simulink library "filters_lib"  (R2018b)
settings: Solver=VariableStepAuto  StartTime=0.0  StopTime=10.0  RelTol=1e-3
undefined symbols (not defined in the file or in its folder): DiscIntNeverNeededParam, u_Trim
libraries: quatAttitudeController_lib x1
settings Model: Creator=Ybeyer  LastModifiedBy=yannic
settings DebuggingCC: LibraryContextMissingDiagnostic=none
settings SFSimCC: SimUseLocalCustomCode=off
settings RTWCC: RTWUseLocalCustomCode=off
settings CodeAppCC: StateflowObjectComments=on

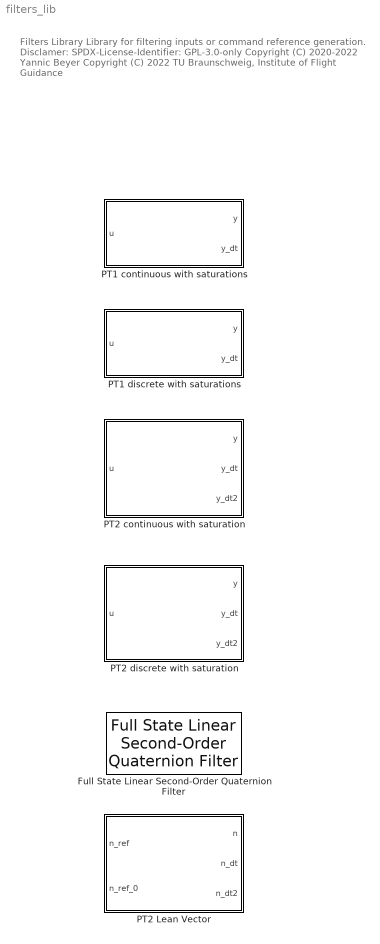
== system filters_lib ==
  note: Filters Library
      |
      | Library for filtering inputs or command reference generation.
      |
      | Disclamer:
      | SPDX-License-Identifier: GPL-3.0-only
      |
      | Copyright (C) 2020-2022 Yannic Beyer
      | Copyright (C) 2022 TU Braunschweig, Institute of Flight Guidance
  Full State Linear Second-Order Quaternion Filter : quatAttitudeController_lib/Full State Linear Second-Order Quaternion Filter  omega_0=15  D=1  q_0=[1; 0; 0; 0]  omega_Kb_0=[0; 0; 0]
      settings: SourceProductName=LADAC
  PT1 continuous with saturations : Subsystem  mask{T=1, x_max=inf, x_min=-inf, x_dt_max=inf, x_dt_min=-inf, x_init=0}
      mask prompts: T "Time constant"; x_max "Maximum output"; x_min "Minimum output"; x_dt_max "Maximum output_rate"; x_dt_min "Minimum output rate"; x_init "Initial output"
  PT1 discrete with saturations : Subsystem  mask{T=1, x_max=inf, x_min=-inf, x_dt_max=inf, x_dt_min=-inf, x_init=u_Trim}
      mask prompts: T "Time constant"; x_max "Maximum output"; x_min "Minimum output"; x_dt_max "Maximum output rate"; x_dt_min "Minimum output rate"; x_init "Initial output"
  PT2 Lean Vector : Subsystem  mask{omega=1, d=1, x_dt2_max=inf, x_dt2_min=-inf, x_dt_max=inf, x_dt_min=-inf, x_max=inf, x_min=-inf, x_init=0, x_dt_init=0}
      mask prompts: omega "Natural frequency"; d "Damping ratio"; x_dt2_max "Maximum acceleration"; x_dt2_min "Minimum acceleration"; x_dt_max "Maximum rate"; x_dt_min "Minimum rate"; x_max "Maximum position"; x_min "Minimum position"; x_init "Initial position"; x_dt_init "Initial rate"
      mask DialogControl DescGroupVar Prompt: 2nd Order Reduced Attitude Reference Model
      mask DialogControl DescTextVar Prompt: The lean vector is filtered by a second order low-pass filter. A unit vector output is assured. Moreover, the derivatives are also adjusted to match with the output unit vector.
  PT2 continuous with saturation : Subsystem  mask{omega=0.7, d=1, x_dt2_max=inf, x_dt2_min=-inf, x_dt_max=inf, x_dt_min=-inf, x_max=inf, x_min=-inf, x_init=0, x_dt_init=0}
      mask prompts: omega "Natural frequency"; d "Damping ratio"; x_dt2_max "Maximum acceleration"; x_dt2_min "Minimum acceleration"; x_dt_max "Maximum rate"; x_dt_min "Minimum rate"; x_max "Maximum position"; x_min "Minimum position"; x_init "Initial position"; x_dt_init "Initial rate"
  PT2 discrete with saturation : Subsystem  mask{param_src=internal, omega=1, d=0.7, x_dt2_max=inf, x_dt2_min=-inf, x_dt_max=inf, x_dt_min=-inf, x_max=inf, x_min=-inf, y_0_src=internal, x_init=0, y_dt_0_src=internal, x_dt_init=0, is_y_dt_checked=on, is_y_dt2_checked=on}
      mask prompts: param_src "Parameter source"; omega "Natural frequency"; d "Damping ratio"; x_dt2_max "Maximum acceleration"; x_dt2_min "Minimum acceleration"; x_dt_max "Maximum rate"; x_dt_min "Minimum rate"; x_max "Maximum position"; x_min "Minimum position"; y_0_src "Initial position source:"; x_init "Initial position"; y_dt_0_src "Initial velocity source:"; x_dt_init "Initial rate"; is_y_dt_checked "Enable velocity output"; is_y_dt2_checked "Enable acceleration output"
      mask init:
      | filtersBlockInit(y_0_src,y_dt_0_src,param_src,is_y_dt_checked,is_y_dt2_checked);
      mask TypeOptions param_src: internal | external
      mask TypeOptions y_0_src: internal | external
      mask TypeOptions y_dt_0_src: internal | external

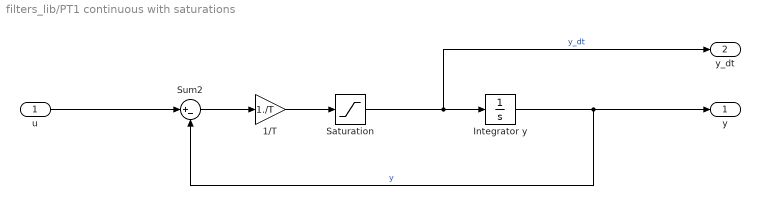
== system filters_lib/PT1 continuous with saturations ==
  u : Inport
  1/T : Gain  Gain=1./T
  Integrator y : Integrator  InitialCondition=x_init  LimitOutput=on  UpperSaturationLimit=x_max  LowerSaturationLimit=x_min
  Saturation : Saturate  UpperLimit=x_dt_max  LowerLimit=x_dt_min
  Sum2 : Sum  Inputs=|+-
  y : Outport
  y_dt : Outport  Port=2
  wires:
  Saturation/1 -> Integrator y/1, y_dt/1  "y_dt"
  Integrator y/1 -> y/1, Sum2/2  "y"
  Sum2/1 -> 1/T/1
  u/1 -> Sum2/1
  1/T/1 -> Saturation/1

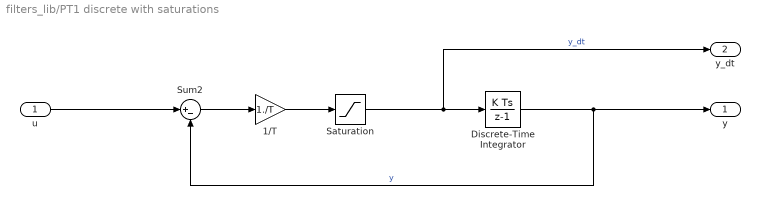
== system filters_lib/PT1 discrete with saturations ==
  u : Inport
  1/T : Gain  Gain=1./T
  Discrete-Time Integrator : DiscreteIntegrator  InitialCondition=x_init  SampleTime=-1  LimitOutput=on  UpperSaturationLimit=x_max  LowerSaturationLimit=x_min  ICPrevOutput=DiscIntNeverNeededParam  ICPrevScaledInput=DiscIntNeverNeededParam
  Saturation : Saturate  UpperLimit=x_dt_max  LowerLimit=x_dt_min
  Sum2 : Sum  Inputs=|+-
  y : Outport
  y_dt : Outport  Port=2
  wires:
  Saturation/1 -> y_dt/1, Discrete-Time Integrator/1  "y_dt"
  Discrete-Time Integrator/1 -> y/1, Sum2/2  "y"
  Sum2/1 -> 1/T/1
  u/1 -> Sum2/1
  1/T/1 -> Saturation/1

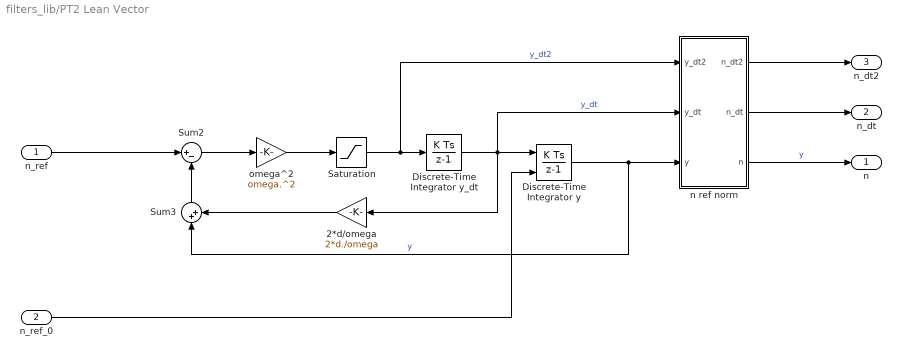
== system filters_lib/PT2 Lean Vector ==
  n_ref : Inport
  n_ref_0 : Inport  Port=2
  2*d/omega : Gain  Gain=2*d./omega
  Discrete-Time Integrator y : DiscreteIntegrator  InitialConditionSource=external  InitialCondition=x_init  SampleTime=-1  OutDataTypeStr=Inherit: Inherit via back propagation  LimitOutput=on  UpperSaturationLimit=x_max  LowerSaturationLimit=x_min  ICPrevOutput=DiscIntNeverNeededParam  ICPrevScaledInput=DiscIntNeverNeededParam
  Discrete-Time Integrator y_dt : DiscreteIntegrator  InitialCondition=x_dt_init  SampleTime=-1  OutDataTypeStr=Inherit: Inherit via back propagation  LimitOutput=on  UpperSaturationLimit=x_dt_max  LowerSaturationLimit=x_dt_min  ICPrevOutput=DiscIntNeverNeededParam  ICPrevScaledInput=DiscIntNeverNeededParam
  Saturation : Saturate  UpperLimit=x_dt2_max  LowerLimit=x_dt2_min
  Sum2 : Sum  Inputs=|+-
  Sum3 : Sum  Inputs=|++
  n ref norm : MATLAB Function  TreatAsAtomicUnit=on
  omega^2 : Gain  Gain=omega.^2
  n : Outport
  n_dt : Outport  Port=2
  n_dt2 : Outport  Port=3
  wires:
  n ref norm/3(n) -> n/1  "y"
  Saturation/1 -> n ref norm/1(y_dt2), Discrete-Time Integrator y_dt/1  "y_dt2"
  omega^2/1 -> Saturation/1
  Sum3/1 -> Sum2/2
  n_ref/1 -> Sum2/1
  2*d/omega/1 -> Sum3/2
  Sum2/1 -> omega^2/1
  Discrete-Time Integrator y/1 -> n ref norm/3(y), Sum3/1  "y"
  Discrete-Time Integrator y_dt/1 -> n ref norm/2(y_dt), 2*d/omega/1, Discrete-Time Integrator y/1  "y_dt"
  n_ref_0/1 -> Discrete-Time Integrator y/2
  n ref norm/1(n_dt2) -> n_dt2/1
  n ref norm/2(n_dt) -> n_dt/1

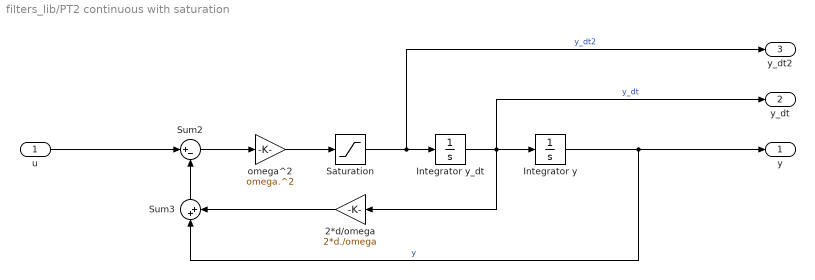
== system filters_lib/PT2 continuous with saturation ==
  u : Inport
  2*d/omega : Gain  Gain=2*d./omega
  Integrator y : Integrator  InitialCondition=x_init  LimitOutput=on  UpperSaturationLimit=x_max  LowerSaturationLimit=x_min
  Integrator y_dt : Integrator  InitialCondition=x_dt_init  LimitOutput=on  UpperSaturationLimit=x_dt_max  LowerSaturationLimit=x_dt_min
  Saturation : Saturate  UpperLimit=x_dt2_max  LowerLimit=x_dt2_min
  Sum2 : Sum  Inputs=|+-
  Sum3 : Sum  Inputs=|++
  omega^2 : Gain  Gain=omega.^2
  y : Outport
  y_dt : Outport  Port=2
  y_dt2 : Outport  Port=3
  wires:
  Integrator y_dt/1 -> y_dt/1, Integrator y/1, 2*d/omega/1  "y_dt"
  Integrator y/1 -> y/1, Sum3/1  "y"
  Sum2/1 -> omega^2/1
  2*d/omega/1 -> Sum3/2
  u/1 -> Sum2/1
  Sum3/1 -> Sum2/2
  omega^2/1 -> Saturation/1
  Saturation/1 -> y_dt2/1, Integrator y_dt/1  "y_dt2"

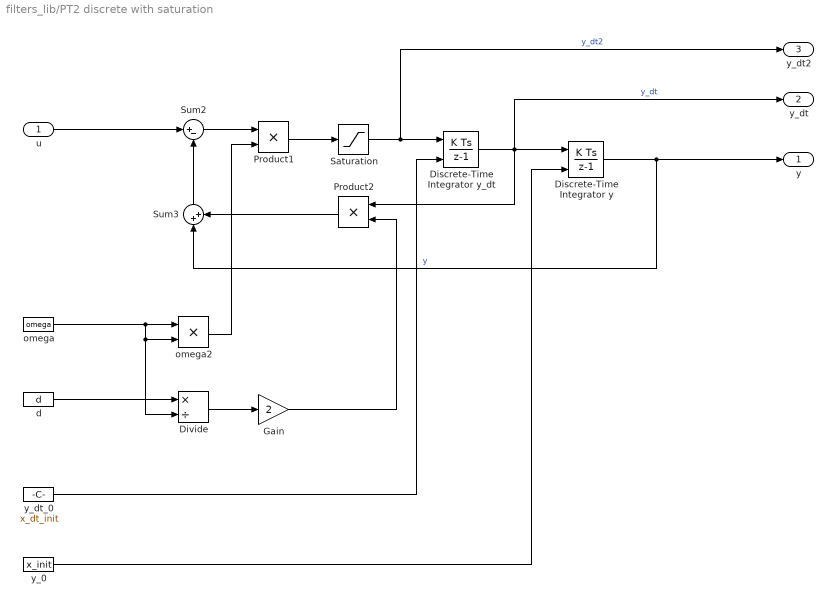
== system filters_lib/PT2 discrete with saturation ==
  u : Inport
  Discrete-Time Integrator y : DiscreteIntegrator  InitialConditionSource=external  InitialCondition=x_init  SampleTime=-1  LimitOutput=on  UpperSaturationLimit=x_max  LowerSaturationLimit=x_min  ICPrevOutput=DiscIntNeverNeededParam  ICPrevScaledInput=DiscIntNeverNeededParam
  Discrete-Time Integrator y_dt : DiscreteIntegrator  InitialConditionSource=external  InitialCondition=x_dt_init  SampleTime=-1  LimitOutput=on  UpperSaturationLimit=x_dt_max  LowerSaturationLimit=x_dt_min  ICPrevOutput=DiscIntNeverNeededParam  ICPrevScaledInput=DiscIntNeverNeededParam
  Divide : Product  Inputs=*/
  Gain : Gain  Gain=2
  Product1 : Product
  Product2 : Product
  Saturation : Saturate  UpperLimit=x_dt2_max  LowerLimit=x_dt2_min
  Sum2 : Sum  Inputs=|+-
  Sum3 : Sum  Inputs=|++
  d : Constant  Value=d
  omega : Constant  Value=omega
  omega2 : Product
  y_0 : Constant  Value=x_init
  y_dt_0 : Constant  Value=x_dt_init
  y : Outport
  y_dt : Outport  Port=2
  y_dt2 : Outport  Port=3
  wires:
  Discrete-Time Integrator y_dt/1 -> Product2/1, Discrete-Time Integrator y/1, y_dt/1  "y_dt"
  Discrete-Time Integrator y/1 -> y/1, Sum3/1  "y"
  Sum2/1 -> Product1/1
  Product2/1 -> Sum3/2
  u/1 -> Sum2/1
  Sum3/1 -> Sum2/2
  Product1/1 -> Saturation/1
  Saturation/1 -> Discrete-Time Integrator y_dt/1, y_dt2/1  "y_dt2"
  y_0/1 -> Discrete-Time Integrator y/2
  y_dt_0/1 -> Discrete-Time Integrator y_dt/2
  omega/1 -> Divide/2, omega2/2, omega2/1
  omega2/1 -> Product1/2
  Divide/1 -> Gain/1
  d/1 -> Divide/1
  Gain/1 -> Product2/2

== matlab function filters_lib/PT2 Lean Vector/n ref norm ==
  data: n_dt2 output; n_dt output; y_dt2 input; y_dt input; y input; n output
function [n_dt2,n_dt,n] = fcn(y_dt2, y_dt, y)

norm_n  = norm(y,2);
n       = divideFinite( y, norm_n );

n_dt    = leanVectorNormDeriv(y,y_dt);
n_dt2   = leanVectorNormDeriv2(y,y_dt,y_dt2);

end
